simulink model "PEMWE_Model"  (R2025b)
settings: Solver=FixedStepAuto  StartTime=0.0  StopTime=10.0  FixedStep=0.01  RelTol=1e-3
InitFcn:
  | run_model_calibration
values from neighbouring files (symbols this model uses):
  form_type = 1    [run_model_calibration.m]
  i_lim = i_lim_final    [run_model_calibration.m]
  kinetic_coefs = reshape(arr_coefs', 1, [])    [run_model_calibration.m]
  T_ref = median(calib_T_K)    [calibration_only.m]    (also in run_model_calibration.m = T_ref_final; validation_only.m)
libraries: simulink x1
settings Model: Creator=HenkerZS  LastModifiedBy=HenkerZS

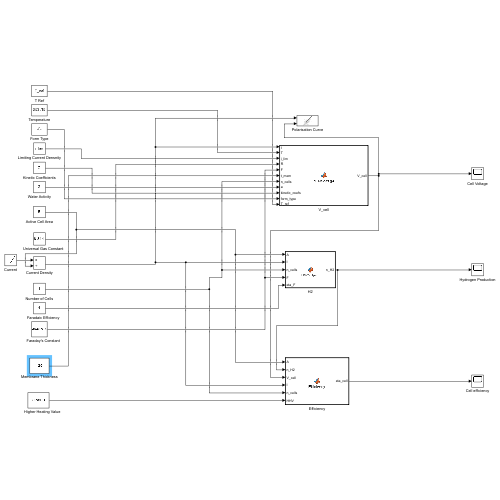
[thumbnail: Simulink's stored preview of the top-level diagram]
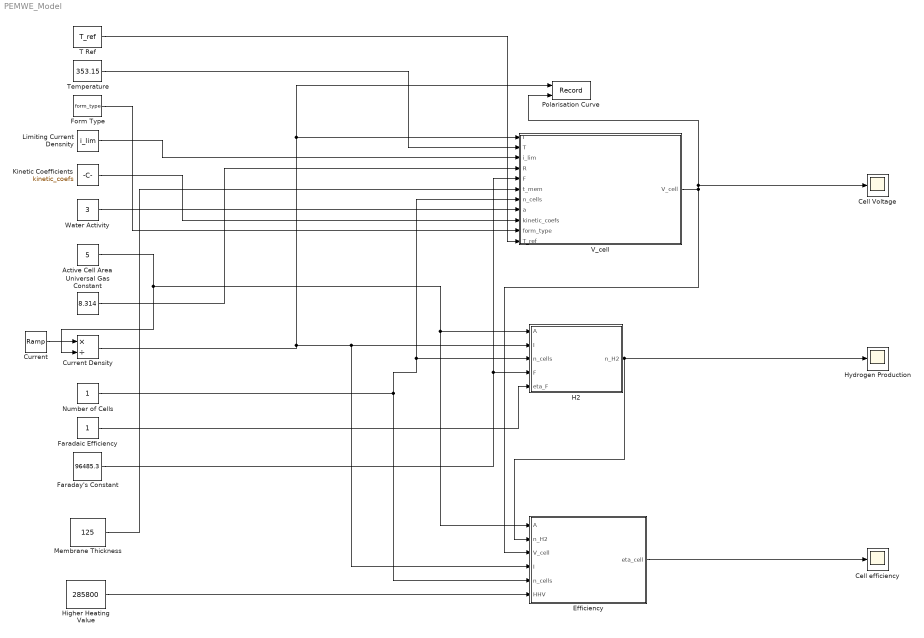
== system PEMWE_Model ==
  "\tFaradaic Efficiency" : Constant
  "\tFaraday's Constant" : Constant  Value=96485.3
  "\tHigher Heating Value" : Constant  Value=285800
  "\tUniversal Gas Constant" : Constant  Value=8.314
  Active Cell Area : Constant  Value=5
  Cell Voltage : Scope
      settings: ActiveDisplayYMinimum=-206.51130651771373  ActiveDisplayYMaximum=1870.3954086594242
  Cell efficiency : Scope
      settings: ActiveDisplayYMinimum=0.62250101738737473  ActiveDisplayYMaximum=1.1666163105231726
  Current : simulink/Sources/Ramp  slope=1  start=0  InitialOutput=0
  Current Density : Product  Inputs=*/
  Efficiency : MATLAB Function  TreatAsAtomicUnit=on
  Form Type : Constant  Value=form_type
  H2 : MATLAB Function  TreatAsAtomicUnit=on
  Hydrogen Production : Scope
      settings: ActiveDisplayYMinimum=-1  ActiveDisplayYMaximum=1  DataLoggingVariableName=ScopeData2
  Kinetic Coefficients : Constant  Value=kinetic_coefs
  Limiting Current Densnity : Constant  Value=i_lim
  Membrane Thickness : Constant  Value=125
  Number of Cells : Constant
  Polarisation Curve : Record  NumPorts=2.0  FileSettingsInternal="{\"entries\":[{\"content\":{\"excelSettings\":{\"content\":{},\"type\":\"Streamout.ExcelSettings\"},\"parquetSettings\":{\"content\":{},\"type\":\"Streamout.ParquetSettings\"}},\"type\":\"Streamout.FileSettingStorage\",\"uuid\":\"\"}],\"packageUris\":[\"http:\\/\\/schema.mathworks.com\\/mf0\\/streamout_blocks\\/R2020a\"],\"version\":\"1.0\"}"  FrameSettings=[0, 0]  Layout=[1 1]  SignalsInternal="{\"entries\":[{\"content\":{\"signals\":[{\"content\":{\"blockPath\":[],\"dimensions\":[1],\"domain\":\"\",\"lineColor\":\"#a2142f\",\"plots\":[ 1 ],\"port\":1,\"sid\":[\"\"],\"signalID\":1,\"signalName\":\"Current Density\"},\"type\":\"RecordBlkView.Signal\",\"uuid\":\"\"},{\"content\":{\"blockPath\":[],\"dimensions\":[1],\"domain\":\"\",\"lineColor\":\"#139fff\",\"plots\":[ 1 ],\"port\":2,\"sid\":[\"\"],\"signalID\":2,\"signalName\":\"V_cell\"},\"type\":\"RecordBlkView.Signal\",\"uuid\":\"\"}]},\"type\":\"RecordBlkView.InputSignals\",\"uuid\":\"\"}],\"packageUris\":[\"http:\\/\\/schema.mathworks.com\\/mf0\\/streamout_blocks\\/R2020a\"],\"version\":\"1.0\"}"  VisualizationBindings="{\"xyplotplugin\":{\"info\":[{\"series\":[{\"bindingParametersList\":[{\"parameter\":\"X-Axis\",\"signalID\":1,\"signalName\":\"Current Density\"},{\"parameter\":\"Y-Axis\",\"signalID\":2,\"signalName\":\"V_cell\"}],\"seriesID\":0}],\"subplotID\":1}]}}"  CompatibilityTag=XY
  T Ref : Constant  Value=T_ref
  Temperature : Constant  Value=353.15
  V_cell : MATLAB Function  TreatAsAtomicUnit=on
  Water Activity : Constant  Value=3
  wires:
  Current/1 -> Current Density/1
  Membrane Thickness/1 -> V_cell/6(t_mem)
  Temperature/1 -> V_cell/2(T)
  "\tUniversal Gas Constant"/1 -> V_cell/4(R)
  "\tFaraday's Constant"/1 -> V_cell/5(F), H2/4(F)
  Number of Cells/1 -> Efficiency/5(n_cells), V_cell/7(n_cells), H2/3(n_cells)
  "\tFaradaic Efficiency"/1 -> H2/5(eta_F)
  "\tHigher Heating Value"/1 -> Efficiency/6(HHV)
  H2/1(n_H2) -> Hydrogen Production/1, Efficiency/2(n_H2)
  V_cell/1(V_cell) -> Polarisation Curve/2, Cell Voltage/1, Efficiency/3(V_cell)
  Efficiency/1(eta_cell) -> Cell efficiency/1
  Current Density/1 -> Polarisation Curve/1, V_cell/1(I), Efficiency/4(I), H2/2(I)
  Active Cell Area/1 -> Current Density/2, Efficiency/1(A), H2/1(A)
  Water Activity/1 -> V_cell/8(a)
  Kinetic Coefficients/1 -> V_cell/9(kinetic_coefs)
  Limiting Current Densnity/1 -> V_cell/3(i_lim)
  Form Type/1 -> V_cell/10(form_type)
  T Ref/1 -> V_cell/11(T_ref)

== matlab function PEMWE_Model/H2 ==
  data: A input; I input; n_H2 output; n_cells input; F input; eta_F input
function n_H2 = H2Output(A, I, n_cells, F, eta_F)
    n_H2 = n_cells * I*A* eta_F / (2*F);   % mol/s
end

== matlab function PEMWE_Model/V_cell ==
  data: I input; V_cell output; T input; i_lim input; R input; F input; t_mem input; n_cells input; a input; kinetic_coefs input; form_type input; T_ref input
function V_cell  = PEMVoltage(I, T, i_lim, R, F, t_mem, n_cells, a, kinetic_coefs, form_type, T_ref)
%PEMVOLTAGE  Steady-state PEM electrolyser single-cell voltage model.
%
%   i_lim, kinetic_coefs, form_type, and T_ref are INPUTS to this block
%   -- they come from Constant blocks in Simulink, each one pointed at
%   a workspace variable name (not a literal number). Those variables
%   are set automatically by run_model_calibration.m, which runs once
%   every time you press Run, via Simulink's InitFcn callback (Model
%   Settings -> Callbacks -> InitFcn -> run_model_calibration).
%
%   WHY NOT calibrate inside this block directly: MATLAB Function
%   blocks are always analysed as if for code generation, even during
%   plain simulation, and readtable/file I/O and fminsearch-based
%   fitting are not supported in that restricted environment. The
%   calibration genuinely has to happen outside this block.
%
%   kinetic_coefs layout:
%     [1] alpha_a coef1   [2] alpha_a coef2
%     [3] alpha_c coef1   [4] alpha_c coef2
%     [5] j0_a coef1      [6] j0_a coef2
%     [7] j0_c coef1      [8] j0_c coef2
%   form_type: 0 = linear, 1 = Arrhenius

    Vrev = 1.229 - 0.9e-3*(T - 298);

    aa_c1 = kinetic_coefs(1); aa_c2 = kinetic_coefs(2);
    ac_c1 = kinetic_coefs(3); ac_c2 = kinetic_coefs(4);
    j0a_c1 = kinetic_coefs(5); j0a_c2 = kinetic_coefs(6);
    j0c_c1 = kinetic_coefs(7); j0c_c2 = kinetic_coefs(8);

    if form_type == 0
        alpha_a = aa_c1*T + aa_c2;
        alpha_c = ac_c1*T + ac_c2;
        j0_a    = j0a_c1*T + j0a_c2;
        j0_c    = j0c_c1*T + j0c_c2;
    else
        alpha_a = aa_c1  * exp(-aa_c2/R  * (1/T - 1/T_ref));
        alpha_c = ac_c1  * exp(-ac_c2/R  * (1/T - 1/T_ref));
        j0_a    = j0a_c1 * exp(-j0a_c2/R * (1/T - 1/T_ref));
        j0_c    = j0c_c1 * exp(-j0c_c2/R * (1/T - 1/T_ref));
    end

    % --- Membrane water content & conductivity (Springer et al., 1991) ---
    a_c = min(max(a, 0), 3);
    if a_c <= 1
        lambda = 0.043 + 17.81*a_c - 39.85*a_c^2 + 36.0*a_c^3;
    else
        lambda = 14 + 1.4*(a_c - 1);
    end
    sigma_raw = (0.005139*lambda - 0.00326) * exp(1268*(1/303 - 1/T));
    sigma = max(sigma_raw, 1e-6);

    eta_act  = 0;
    eta_ohm  = 0;
    eta_diff = 0;

    if I > 0
        eta_act = (R*T/(alpha_a*F)) * asinh(I/(2*j0_a)) + ...
                  (R*T/(alpha_c*F)) * asinh(I/(2*j0_c));
        eta_ohm = I * (t_mem/sigma);
        i_safe   = min(I, 0.999*i_lim);
        eta_diff = (R*T/F) * log(i_lim/(i_lim - i_safe));
    end

    V_cell = Vrev + eta_act + eta_ohm + eta_diff;
end

== matlab function PEMWE_Model/Efficiency ==
  data: A input; n_H2 input; eta_cell output; V_cell input; I input; n_cells input; HHV input
function eta_cell = Efficiency(A,n_H2, V_cell, I, n_cells, HHV)
    P_in = n_cells * V_cell * I*A;
    eta_cell = (n_H2 * HHV) / P_in;
end
